simulink model "EMT"  (R2024b)
settings: Solver=ode5  StartTime=0.0  StopTime=1500  FixedStep=0.002  RelTol=1e-3
PreLoadFcn:
  | parameter;
InitFcn:
  | parameter;
StopFcn:
  | save('result.mat');
values from neighbouring files (symbols this model uses):
  A = 7.3    [parameter.m]
  a11 = (1+k1)*(1+k2)/k1/k2/iq    (= 1.54241568346)    [parameter.m]
  a11_L = a11    (= 1.54241568346)    [parameter.m]
  a12 = -(1+k1+k2)*(1+k3)/k1/k2    (= -3.86074191629)    [parameter.m]
  a12_L = a11*(1+k3+k4)/(1+k3)    (= 2.43173643789)    [parameter.m]
  a21 = -(1+k2)/k1/iq    (= -1.04963112005)    [parameter.m]
  a22 = (1+k1+k2)/k1    (= 2.46948356808)    [parameter.m]
  B = 2.71    [parameter.m]
  b11 = 0    [parameter.m]
  b12 = (1+k3)    (= 3.33)    [parameter.m]
  b21 = (1+k2)/iq    (= 2.23571428571)    [parameter.m]
  b22 = -k2    (= -2.13)    [parameter.m]
  C1_shift = 200    [parameter.m]
  Cb = 70    [parameter.m]
  Cd = 0.6    [parameter.m]
  eff_generator = eff_motor    [parameter.m]
  eff_motor = [0.80 0.80 0.84 0.84 0.83 0.85 0.83 0.83 0.83 0.80 0.80 0.80 ... (first row only)    [parameter.m]
  ele_map = [10.00,11.46,14.13,19.24,20.94,23.21,20.29,20.23,22.28,17.66,16.24,18.95,20.79,16.98,18.22,16.52,18.29,20.67,20.82,23.14,23.36,21.30,17.71,20.26,19.53,21.18,23.13,22.79,19.35,16.77,20.50,19.02,20.56,21.90,23.91,20.40,18.45,22.70,22.38,22.48,21.84,17.76,20.13,22.61,19.35,19.36,21.56,20.37,18.38,17.96,18.38,17.24,18.99,22.31,23.50,18.24,22.11,20.73,20.35,18.91,22.88,20.92,18.75,16.85,21.94,17.80,19. ...(+2007 chars)    [parameter.m]
  Fb_max = 5.5*mass    (= 247500)    [parameter.m]
  ic = 4.42    [parameter.m]
  JA = 0.4    [parameter.m]
  JB = JA    (= 0.4)    [parameter.m]
  Jc3r4 = 1e-2    (= 0.01)    [parameter.m]
  Je = 2.5    [parameter.m]
  Jh = 1e-2    (= 0.01)    [parameter.m]
  kh = 2.88    [parameter.m]
  kt = 1.83    [parameter.m]
  L = 4.472    [parameter.m]
  mass = 45000    [parameter.m]
  miu_max = 0.8    [parameter.m]
  n_generator = n_motor    [parameter.m]
  n_motor = [0 0.1 0.25 0.4 0.55 0.7 0.85 1 1.15 1.3 1.45 2.2]*3185    [parameter.m]
  nA_map = [-6000:50:-3250 -3200 0 3200 3250:50:6000]    [parameter.m]    (also in plot_result.m = [-7000:50:-3250 -3200 0 3200 3250:50:7000])
  nA_max = max(nA_map)    [parameter.m]
  nA_min = min(nA_map)    [parameter.m]
  nB_map = nA_map    [parameter.m]    (also in plot_result.m = [-7000:50:-3250 -3200 0 3200 3250:50:7000])
  nB_max = nA_max    [parameter.m]
  nB_min = nA_min    [parameter.m]
  ne_idl = 3000    [parameter.m]
  ne_map = [1600,1700,1800,1900,2000,2100,2200,2300,2400,2500,2600,2700,2800,2900,3000,3100,3200,3300,3400,3500,3600,3700,3800,3900,4000,4100,4200,4500]    [parameter.m]
  ne_max = 4200    [parameter.m]
  ne_min = 1600    [parameter.m]
  ne_start = 200    [parameter.m]
  nZ_map = [-8000:50:-4850 -4800 0 4800 4850:50:8000]    [parameter.m]
  Pb_epr = [-45 -45 -40 -30 0 30 40 45 45]    [parameter.m]
  Pb_max = [0 40 45 45 45]    [parameter.m]
  Pb_min = [-45 -45 -45 -40 0]    [parameter.m]
  Pe_ass = 210+20    (= 230)    [parameter.m]
  Pe_max = 1103    [parameter.m]
  PN0 = 0    [parameter.m]
  R_map = [0.90 0.89 0.90 0.91 0.92 0.93 0.94 0.95 0.96 0.97 0.98]/10    [parameter.m]
  rz = 0.318    [parameter.m]
  SOC0 = 60    [parameter.m]
  SOC_epr = [30 31 50 59 60 61 70 79 80]    [parameter.m]
  SOC_map = 0:10:100    [parameter.m]
  T_generator = T_motor    [parameter.m]
  T_motor = [0 0.3 0.8 1.3 1.8 2.3 2.8]/1.8*1110    [parameter.m]
  TA_max_map = [370*9549./(6000:-50:3250) 1110 1110 1110 370*9549./(3250:50:6000)]    [parameter.m]    (also in plot_result.m = [370*9549./(7000:-50:3250) 1100 1100 1100 370*9549./(3250:50)
  TA_min_map = -TA_max_map    [parameter.m]
  TAf = 0    [parameter.m]
  TB_max_map = TA_max_map    [parameter.m]    (also in plot_result.m = [370*9549./(7000:-50:3250) 1110 1110 1110 370*9549./(3250:50)
  TB_min_map = TA_min_map    [parameter.m]
  TBf = TAf    (= 0)    [parameter.m]
  Te_map = [0,599,798,998,1168,1324,1495,1660,1822,1970,2106,2235,2355,2458,2508,2543,2565,2606,2613,2649,2658,2689,2701,2707,2719,2724,2728,2740,2743,2754]    [parameter.m]
  Te_max_map = [1168,1324,1495,1660,1822,1970,2106,2235,2355,2458,2543,2606,2658,2701,2728,2743,2754,2743,2740,2724,2719,2707,2689,2649,2613,2565,2508,998]    [parameter.m]
  Te_start = 1600    [parameter.m]
  Tef = 100    [parameter.m]
  Time = 0:0.1:200    [parameter.m]
  Time_ele = 0:4:1600    [parameter.m]
  TS_A = 0.2    [parameter.m]
  TS_B = TS_A    (= 0.2)    [parameter.m]
  TS_C0 = 0.2    [parameter.m]
  TS_C1 = 0.2    [parameter.m]
  Ts_e = 0.1    [parameter.m]
  TS_Z1 = 0.2    [parameter.m]
  TS_Z2 = 0.2    [parameter.m]
  TZ_max_map = [450*9549./(8000:-50:4850) 1000 1000 1000 450*9549./(4850:50:8000)]    [parameter.m]
  TZ_min_map = -TZ_max_map    [parameter.m]
  Uoc_map = [3.258,3.668,3.733,3.783,3.833,3.877,3.912,3.941,3.973,4.013,4.200]*250    [parameter.m]
  v_cyc = 0.*(0<=Time&Time<11)+(3.75.*Time-41.25).*(11<=Time&Time<15)+15.*(15<=Time&Time<23)+(-3.*Time+84).*(23<=Time&Time<28)+0.*(28<=Time&Time<49)+(8.*Time/3-392/3).*(49<=Time&Time<61)+32.*(61<=Time&Time<85)+(-32.*Time/11+3072/11).*(85<=Time&Time<96)+0.*(96<=Time&Time<117)+(25.*Time/13-2925/13).*(117<=Time&Time<143)+50.*(143<=Time&Time<155)+(-15.*Time/8+2725/8).*(155<=Time&Time<163)+35.*(163<=Time&Time<17 ...(+70 chars)    [parameter.m]
  V_Shift12 = 32    [parameter.m]
  V_Shift21 = 25    [parameter.m]
  Voltage_epr = [750 760 900 1000 1050]    [parameter.m]
  Y_engine = 0.955    [parameter.m]
  Yc = 0.98    [parameter.m]
  Yh = 0.96    [parameter.m]
  Z1_shift = 200    [parameter.m]
  Z2_shift = 200    [parameter.m]
undefined symbols (not defined in the file or in its folder): sigbuilder_block
libraries: fl_lib x82, nesl_utility x55, simulink x49, sdl_lib x10, simulink_need_slupdate x6, powerlib_extras x1
(part 5 of 6)

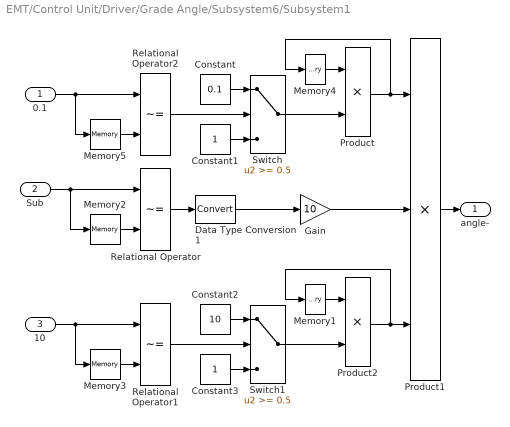
== system EMT/Control Unit/Driver/Grade Angle/Subsystem6/Subsystem1 ==
  0.1 : Inport
  Sub : Inport  Port=2
  10 : Inport  Port=3
  Constant : Constant  Value=0.1
  Constant1 : Constant
  Constant2 : Constant  Value=10
  Constant3 : Constant
  Data Type Conversion1 : DataTypeConversion  SaturateOnIntegerOverflow=off  RndMeth=Floor
  Gain : Gain  Gain=10
  Memory1 : Memory  InitialCondition=1
  Memory2 : Memory
  Memory3 : Memory
  Memory4 : Memory  InitialCondition=1
  Memory5 : Memory
  Product : Product  RndMeth=Zero
  Product1 : Product  Inputs=3  RndMeth=Zero
  Product2 : Product  RndMeth=Zero
  Relational Operator : RelationalOperator  Operator=~=  OutDataTypeStr=boolean  InputSameDT=off
  Relational Operator1 : RelationalOperator  Operator=~=  OutDataTypeStr=boolean  InputSameDT=off
  Relational Operator2 : RelationalOperator  Operator=~=  OutDataTypeStr=boolean  InputSameDT=off
  Switch : Switch  Threshold=0.5  SaturateOnIntegerOverflow=off  InputSameDT=off
  Switch1 : Switch  Threshold=0.5  SaturateOnIntegerOverflow=off  InputSameDT=off
  angle- : Outport
  wires:
  Switch1/1 -> Product2/2
  Constant3/1 -> Switch1/3
  Constant2/1 -> Switch1/1
  10/1 -> Memory3/1, Relational Operator1/1
  Relational Operator1/1 -> Switch1/2
  Memory3/1 -> Relational Operator1/2
  Memory1/1 -> Product2/1
  Product2/1 -> Product1/3, Memory1/1
  Product1/1 -> angle-/1
  Switch/1 -> Product/2
  Constant1/1 -> Switch/3
  Constant/1 -> Switch/1
  0.1/1 -> Relational Operator2/1, Memory5/1
  Relational Operator2/1 -> Switch/2
  Memory5/1 -> Relational Operator2/2
  Memory4/1 -> Product/1
  Product/1 -> Product1/1, Memory4/1
  Data Type Conversion1/1 -> Gain/1
  Relational Operator/1 -> Data Type Conversion1/1
  Sub/1 -> Memory2/1, Relational Operator/1
  Memory2/1 -> Relational Operator/2
  Gain/1 -> Product1/2

== system EMT/Control Unit/Driver/Ground Resistance Coefficient/Road/Subsystem ==
  In : Inport
  Add : Sum  Inputs=+++
  Compare To Constant1 : simulink/Logic and Bit Operations/Compare To Constant  relop=>  const=0.01  OutDataTypeStr=uint8
  Compare To Constant2 : simulink/Logic and Bit Operations/Compare To Constant  relop=>  const=0.2  OutDataTypeStr=uint8
  Compare To Constant3 : simulink/Logic and Bit Operations/Compare To Constant  relop=>  const=0.8  OutDataTypeStr=uint8
  Compare To Constant4 : simulink/Logic and Bit Operations/Compare To Constant  relop=<  const=1  OutDataTypeStr=uint8
  Data Type Conversion : DataTypeConversion  SaturateOnIntegerOverflow=off  RndMeth=Floor
  Logical Operator1 : Logic  Operator=OR  AllPortsSameDT=off  OutDataTypeStr=boolean
  Memory2 : Memory
  Judge : Outport
  wires:
  Compare To Constant2/1 -> Add/2
  Data Type Conversion/1 -> Judge/1
  Compare To Constant1/1 -> Add/1
  Add/1 -> Data Type Conversion/1
  In/1 -> Compare To Constant3/1, Compare To Constant2/1, Compare To Constant1/1
  [v_act] -> Memory2/1
  Memory2/1 -> Compare To Constant4/1
  Compare To Constant4/1 -> Logical Operator1/2
  Compare To Constant3/1 -> Logical Operator1/1
  Logical Operator1/1 -> Add/3

== system EMT/Control Unit/Driver/Ground Resistance Coefficient/Road/Subsystem1 ==
  Constant5 : Constant  Value=0.6
  Out1 : Outport
  wires:
  Constant5/1 -> Out1/1

== system EMT/Control Unit/Driver/Ground Resistance Coefficient/Road/Subsystem2 ==
  In1 : Inport
  1-D Lookup Table : Lookup_n-D  NumberOfTableDimensions=1  BreakpointsForDimension1=[-1 0 0.1 0.2 0.8 1]  Table=[0.6 0.1 0.04 0 0 0]  RndMeth=Simplest
  Saturation : Saturate  UpperLimit=1  LowerLimit=-1
  Out1 : Outport
  wires:
  Saturation/1 -> 1-D Lookup Table/1
  In1/1 -> Saturation/1
  1-D Lookup Table/1 -> Out1/1

== system EMT/Control Unit/Driver/Ground Resistance Coefficient/Road/Subsystem3 ==
  Constant1 : Constant  Value=0
  Out1 : Outport
  wires:
  Constant1/1 -> Out1/1

== system EMT/Control Unit/Driver/Ground Resistance Coefficient/Road/Subsystem4 ==
  Constant1 : Constant  Value=-0.04
  Out1 : Outport
  wires:
  Constant1/1 -> Out1/1

== system EMT/Control Unit/Driver/Ground Resistance Coefficient/Subsystem2/Subsystem4 ==
  11 : Constant
  21 : Constant  Value=2
  22 : Constant  Value=3
  31 : Constant  Value=4
  0.1 : Outport
  0.01 : Outport  Port=2
  10 : Outport  Port=3
  100 : Outport  Port=4
  wires:
  11/1 -> 0.1/1
  21/1 -> 0.01/1
  22/1 -> 10/1
  31/1 -> 100/1

== system EMT/Control Unit/Driver/Ground Resistance Coefficient/Subsystem2/Subsystem6 ==
  11 : Constant
  21 : Constant  Value=2
  22 : Constant  Value=3
  31 : Constant  Value=4
  1 : Outport
  2 : Outport  Port=2
  3 : Outport  Port=3
  4 : Outport  Port=4
  wires:
  31/1 -> 4/1
  22/1 -> 3/1
  21/1 -> 2/1
  11/1 -> 1/1

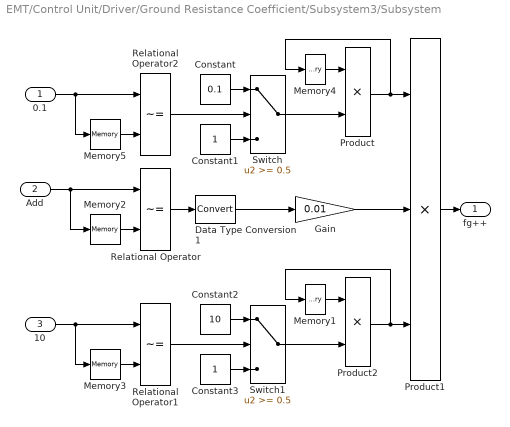
== system EMT/Control Unit/Driver/Ground Resistance Coefficient/Subsystem3/Subsystem ==
  0.1 : Inport
  Add : Inport  Port=2
  10 : Inport  Port=3
  Constant : Constant  Value=0.1
  Constant1 : Constant
  Constant2 : Constant  Value=10
  Constant3 : Constant
  Data Type Conversion1 : DataTypeConversion  SaturateOnIntegerOverflow=off  RndMeth=Floor
  Gain : Gain  Gain=0.01
  Memory1 : Memory  InitialCondition=1
  Memory2 : Memory
  Memory3 : Memory
  Memory4 : Memory  InitialCondition=1
  Memory5 : Memory
  Product : Product  RndMeth=Zero
  Product1 : Product  Inputs=3  RndMeth=Zero
  Product2 : Product  RndMeth=Zero
  Relational Operator : RelationalOperator  Operator=~=  OutDataTypeStr=boolean  InputSameDT=off
  Relational Operator1 : RelationalOperator  Operator=~=  OutDataTypeStr=boolean  InputSameDT=off
  Relational Operator2 : RelationalOperator  Operator=~=  OutDataTypeStr=boolean  InputSameDT=off
  Switch : Switch  Threshold=0.5  SaturateOnIntegerOverflow=off  InputSameDT=off
  Switch1 : Switch  Threshold=0.5  SaturateOnIntegerOverflow=off  InputSameDT=off
  fg++ : Outport
  wires:
  Gain/1 -> Product1/2
  Switch1/1 -> Product2/2
  Constant3/1 -> Switch1/3
  Constant2/1 -> Switch1/1
  10/1 -> Memory3/1, Relational Operator1/1
  Relational Operator1/1 -> Switch1/2
  Memory3/1 -> Relational Operator1/2
  Memory1/1 -> Product2/1
  Product2/1 -> Product1/3, Memory1/1
  Product1/1 -> fg++/1
  Switch/1 -> Product/2
  Constant1/1 -> Switch/3
  Constant/1 -> Switch/1
  0.1/1 -> Relational Operator2/1, Memory5/1
  Relational Operator2/1 -> Switch/2
  Memory5/1 -> Relational Operator2/2
  Memory4/1 -> Product/1
  Product/1 -> Product1/1, Memory4/1
  Data Type Conversion1/1 -> Gain/1
  Relational Operator/1 -> Data Type Conversion1/1
  Add/1 -> Memory2/1, Relational Operator/1
  Memory2/1 -> Relational Operator/2

== system EMT/Control Unit/Driver/Ground Resistance Coefficient/Subsystem3/Subsystem1 ==
  0.1 : Inport
  Sub : Inport  Port=2
  10 : Inport  Port=3
  Constant : Constant  Value=0.1
  Constant1 : Constant
  Constant2 : Constant  Value=10
  Constant3 : Constant
  Data Type Conversion1 : DataTypeConversion  SaturateOnIntegerOverflow=off  RndMeth=Floor
  Gain : Gain  Gain=0.01
  Memory1 : Memory  InitialCondition=1
  Memory2 : Memory
  Memory3 : Memory
  Memory4 : Memory  InitialCondition=1
  Memory5 : Memory
  Product : Product  RndMeth=Zero
  Product1 : Product  Inputs=3  RndMeth=Zero
  Product2 : Product  RndMeth=Zero
  Relational Operator : RelationalOperator  Operator=~=  OutDataTypeStr=boolean  InputSameDT=off
  Relational Operator1 : RelationalOperator  Operator=~=  OutDataTypeStr=boolean  InputSameDT=off
  Relational Operator2 : RelationalOperator  Operator=~=  OutDataTypeStr=boolean  InputSameDT=off
  Switch : Switch  Threshold=0.5  SaturateOnIntegerOverflow=off  InputSameDT=off
  Switch1 : Switch  Threshold=0.5  SaturateOnIntegerOverflow=off  InputSameDT=off
  fg-- : Outport
  wires:
  Gain/1 -> Product1/2
  Memory2/1 -> Relational Operator/2
  Sub/1 -> Relational Operator/1, Memory2/1
  Relational Operator/1 -> Data Type Conversion1/1
  Data Type Conversion1/1 -> Gain/1
  Product/1 -> Memory4/1, Product1/1
  Memory4/1 -> Product/1
  Memory5/1 -> Relational Operator2/2
  Relational Operator2/1 -> Switch/2
  0.1/1 -> Memory5/1, Relational Operator2/1
  Constant/1 -> Switch/1
  Constant1/1 -> Switch/3
  Switch/1 -> Product/2
  Product1/1 -> fg--/1
  Product2/1 -> Memory1/1, Product1/3
  Memory1/1 -> Product2/1
  Memory3/1 -> Relational Operator1/2
  Relational Operator1/1 -> Switch1/2
  10/1 -> Relational Operator1/1, Memory3/1
  Constant2/1 -> Switch1/1
  Constant3/1 -> Switch1/3
  Switch1/1 -> Product2/2

== system EMT/Control Unit/Driver/Pedal /Subsystem13/Subsystem4 ==
  11 : Constant
  21 : Constant  Value=2
  22 : Constant  Value=3
  31 : Constant  Value=4
  0.1 : Outport
  0.01 : Outport  Port=2
  10 : Outport  Port=3
  100 : Outport  Port=4
  wires:
  31/1 -> 100/1
  22/1 -> 10/1
  21/1 -> 0.01/1
  11/1 -> 0.1/1

== system EMT/Control Unit/Driver/Pedal /Subsystem13/Subsystem6 ==
  11 : Constant
  21 : Constant  Value=2
  22 : Constant  Value=3
  31 : Constant  Value=4
  1 : Outport
  2 : Outport  Port=2
  3 : Outport  Port=3
  4 : Outport  Port=4
  wires:
  11/1 -> 1/1
  21/1 -> 2/1
  22/1 -> 3/1
  31/1 -> 4/1

== system EMT/Control Unit/Driver/Pedal /Subsystem5/Subsystem ==
  0.1 : Inport
  Add : Inport  Port=2
  10 : Inport  Port=3
  Constant : Constant  Value=0.1
  Constant1 : Constant
  Constant2 : Constant  Value=10
  Constant3 : Constant
  Data Type Conversion1 : DataTypeConversion  SaturateOnIntegerOverflow=off  RndMeth=Floor
  Gain : Gain  Gain=0.1
  Memory1 : Memory  InitialCondition=1
  Memory2 : Memory
  Memory3 : Memory
  Memory4 : Memory  InitialCondition=1
  Memory5 : Memory
  Product : Product  RndMeth=Zero
  Product1 : Product  Inputs=3  RndMeth=Zero
  Product2 : Product  RndMeth=Zero
  Relational Operator : RelationalOperator  Operator=~=  OutDataTypeStr=boolean  InputSameDT=off
  Relational Operator1 : RelationalOperator  Operator=~=  OutDataTypeStr=boolean  InputSameDT=off
  Relational Operator2 : RelationalOperator  Operator=~=  OutDataTypeStr=boolean  InputSameDT=off
  Switch : Switch  Threshold=0.5  SaturateOnIntegerOverflow=off  InputSameDT=off
  Switch1 : Switch  Threshold=0.5  SaturateOnIntegerOverflow=off  InputSameDT=off
  pedal++ : Outport
  wires:
  Memory2/1 -> Relational Operator/2
  Add/1 -> Relational Operator/1, Memory2/1
  Relational Operator/1 -> Data Type Conversion1/1
  Data Type Conversion1/1 -> Gain/1
  Product/1 -> Memory4/1, Product1/1
  Memory4/1 -> Product/1
  Memory5/1 -> Relational Operator2/2
  Relational Operator2/1 -> Switch/2
  0.1/1 -> Memory5/1, Relational Operator2/1
  Constant/1 -> Switch/1
  Constant1/1 -> Switch/3
  Switch/1 -> Product/2
  Product1/1 -> pedal++/1
  Product2/1 -> Memory1/1, Product1/3
  Memory1/1 -> Product2/1
  Memory3/1 -> Relational Operator1/2
  Relational Operator1/1 -> Switch1/2
  10/1 -> Relational Operator1/1, Memory3/1
  Constant2/1 -> Switch1/1
  Constant3/1 -> Switch1/3
  Switch1/1 -> Product2/2
  Gain/1 -> Product1/2

== system EMT/Control Unit/Driver/Pedal /Subsystem5/Subsystem1 ==
  0.1 : Inport
  Sub : Inport  Port=2
  10 : Inport  Port=3
  Constant : Constant  Value=0.1
  Constant1 : Constant
  Constant2 : Constant  Value=10
  Constant3 : Constant
  Data Type Conversion1 : DataTypeConversion  SaturateOnIntegerOverflow=off  RndMeth=Floor
  Gain : Gain  Gain=0.1
  Memory1 : Memory  InitialCondition=1
  Memory2 : Memory
  Memory3 : Memory
  Memory4 : Memory  InitialCondition=1
  Memory5 : Memory
  Product : Product  RndMeth=Zero
  Product1 : Product  Inputs=3  RndMeth=Zero
  Product2 : Product  RndMeth=Zero
  Relational Operator : RelationalOperator  Operator=~=  OutDataTypeStr=boolean  InputSameDT=off
  Relational Operator1 : RelationalOperator  Operator=~=  OutDataTypeStr=boolean  InputSameDT=off
  Relational Operator2 : RelationalOperator  Operator=~=  OutDataTypeStr=boolean  InputSameDT=off
  Switch : Switch  Threshold=0.5  SaturateOnIntegerOverflow=off  InputSameDT=off
  Switch1 : Switch  Threshold=0.5  SaturateOnIntegerOverflow=off  InputSameDT=off
  pedal-- : Outport
  wires:
  Switch1/1 -> Product2/2
  Constant3/1 -> Switch1/3
  Constant2/1 -> Switch1/1
  10/1 -> Memory3/1, Relational Operator1/1
  Relational Operator1/1 -> Switch1/2
  Memory3/1 -> Relational Operator1/2
  Memory1/1 -> Product2/1
  Product2/1 -> Product1/3, Memory1/1
  Product1/1 -> pedal--/1
  Switch/1 -> Product/2
  Constant1/1 -> Switch/3
  Constant/1 -> Switch/1
  0.1/1 -> Relational Operator2/1, Memory5/1
  Relational Operator2/1 -> Switch/2
  Memory5/1 -> Relational Operator2/2
  Memory4/1 -> Product/1
  Product/1 -> Product1/1, Memory4/1
  Data Type Conversion1/1 -> Gain/1
  Relational Operator/1 -> Data Type Conversion1/1
  Sub/1 -> Memory2/1, Relational Operator/1
  Memory2/1 -> Relational Operator/2
  Gain/1 -> Product1/2

== system EMT/Control Unit/Driver/Wheel Angle/Subsystem1/Subsystem4 ==
  11 : Constant
  21 : Constant  Value=2
  22 : Constant  Value=3
  31 : Constant  Value=4
  0.1 : Outport
  0.01 : Outport  Port=2
  10 : Outport  Port=3
  100 : Outport  Port=4
  wires:
  31/1 -> 100/1
  22/1 -> 10/1
  21/1 -> 0.01/1
  11/1 -> 0.1/1

== system EMT/Control Unit/Driver/Wheel Angle/Subsystem1/Subsystem6 ==
  11 : Constant
  21 : Constant  Value=2
  22 : Constant  Value=3
  31 : Constant  Value=4
  1 : Outport
  2 : Outport  Port=2
  3 : Outport  Port=3
  4 : Outport  Port=4
  wires:
  11/1 -> 1/1
  21/1 -> 2/1
  22/1 -> 3/1
  31/1 -> 4/1

== system EMT/Control Unit/Driver/Wheel Angle/Subsystem2/Subsystem ==
  0.1 : Inport
  Add : Inport  Port=2
  10 : Inport  Port=3
  Constant : Constant  Value=0.1
  Constant1 : Constant
  Constant2 : Constant  Value=10
  Constant3 : Constant
  Data Type Conversion1 : DataTypeConversion  SaturateOnIntegerOverflow=off  RndMeth=Floor
  Gain : Gain
  Memory1 : Memory  InitialCondition=1
  Memory2 : Memory
  Memory3 : Memory
  Memory4 : Memory  InitialCondition=1
  Memory5 : Memory
  Product : Product  RndMeth=Zero
  Product1 : Product  Inputs=3  RndMeth=Zero
  Product2 : Product  RndMeth=Zero
  Relational Operator : RelationalOperator  Operator=~=  OutDataTypeStr=boolean  InputSameDT=off
  Relational Operator1 : RelationalOperator  Operator=~=  OutDataTypeStr=boolean  InputSameDT=off
  Relational Operator2 : RelationalOperator  Operator=~=  OutDataTypeStr=boolean  InputSameDT=off
  Switch : Switch  Threshold=0.5  SaturateOnIntegerOverflow=off  InputSameDT=off
  Switch1 : Switch  Threshold=0.5  SaturateOnIntegerOverflow=off  InputSameDT=off
  wheel++ : Outport
  wires:
  Memory2/1 -> Relational Operator/2
  Add/1 -> Relational Operator/1, Memory2/1
  Relational Operator/1 -> Data Type Conversion1/1
  Data Type Conversion1/1 -> Gain/1
  Product/1 -> Memory4/1, Product1/1
  Memory4/1 -> Product/1
  Memory5/1 -> Relational Operator2/2
  Relational Operator2/1 -> Switch/2
  0.1/1 -> Memory5/1, Relational Operator2/1
  Constant/1 -> Switch/1
  Constant1/1 -> Switch/3
  Switch/1 -> Product/2
  Product1/1 -> wheel++/1
  Product2/1 -> Memory1/1, Product1/3
  Memory1/1 -> Product2/1
  Memory3/1 -> Relational Operator1/2
  Relational Operator1/1 -> Switch1/2
  10/1 -> Relational Operator1/1, Memory3/1
  Constant2/1 -> Switch1/1
  Constant3/1 -> Switch1/3
  Switch1/1 -> Product2/2
  Gain/1 -> Product1/2

== system EMT/Control Unit/Driver/Wheel Angle/Subsystem2/Subsystem1 ==
  0.1 : Inport
  Sub : Inport  Port=2
  10 : Inport  Port=3
  Constant : Constant  Value=0.1
  Constant1 : Constant
  Constant2 : Constant  Value=10
  Constant3 : Constant
  Data Type Conversion1 : DataTypeConversion  SaturateOnIntegerOverflow=off  RndMeth=Floor
  Gain : Gain
  Memory1 : Memory  InitialCondition=1
  Memory2 : Memory
  Memory3 : Memory
  Memory4 : Memory  InitialCondition=1
  Memory5 : Memory
  Product : Product  RndMeth=Zero
  Product1 : Product  Inputs=3  RndMeth=Zero
  Product2 : Product  RndMeth=Zero
  Relational Operator : RelationalOperator  Operator=~=  OutDataTypeStr=boolean  InputSameDT=off
  Relational Operator1 : RelationalOperator  Operator=~=  OutDataTypeStr=boolean  InputSameDT=off
  Relational Operator2 : RelationalOperator  Operator=~=  OutDataTypeStr=boolean  InputSameDT=off
  Switch : Switch  Threshold=0.5  SaturateOnIntegerOverflow=off  InputSameDT=off
  Switch1 : Switch  Threshold=0.5  SaturateOnIntegerOverflow=off  InputSameDT=off
  wheel-- : Outport
  wires:
  Switch1/1 -> Product2/2
  Constant3/1 -> Switch1/3
  Constant2/1 -> Switch1/1
  10/1 -> Memory3/1, Relational Operator1/1
  Relational Operator1/1 -> Switch1/2
  Memory3/1 -> Relational Operator1/2
  Memory1/1 -> Product2/1
  Product2/1 -> Product1/3, Memory1/1
  Product1/1 -> wheel--/1
  Switch/1 -> Product/2
  Constant1/1 -> Switch/3
  Constant/1 -> Switch/1
  0.1/1 -> Relational Operator2/1, Memory5/1
  Relational Operator2/1 -> Switch/2
  Memory5/1 -> Relational Operator2/2
  Memory4/1 -> Product/1
  Product/1 -> Product1/1, Memory4/1
  Data Type Conversion1/1 -> Gain/1
  Relational Operator/1 -> Data Type Conversion1/1
  Sub/1 -> Memory2/1, Relational Operator/1
  Memory2/1 -> Relational Operator/2
  Gain/1 -> Product1/2

== system EMT/Power Coupler /Z1/Z/Power/Speed Sensor ==
  Ideal Rotational Motion Sensor : fl_lib/Mechanical/Mechanical Sensors/Ideal Rotational Motion Sensor  reference=foundation.enum.MeasurementReference.difference  acceleration_port=false  velocity_port=true  position_port=true  wrap_angle=false  offset=0 rad
  PS-Simulink Converter : nesl_utility/PS-Simulink Converter  PhysicalDomain=network_engine_domain  SubClassName=ps_output  LeftPortType=input  RightPortType=output  PseudoPeriodic=off  Frequencies=[]  VectorFormat=1-D array  Unit=rad/s  AffineConversion=off
  Reference : fl_lib/Mechanical/Rotational Elements/Mechanical Rotational Reference
  Tire Radius2 : Gain  Gain=30/pi
  shaft : PMIOPort  Side=Left
  r/min : Outport
  wires:
  Tire Radius2/1 -> r/min/1
  PS-Simulink Converter/1 -> Tire Radius2/1
  connections:
  shaft/RConn1 -- Ideal Rotational Motion Sensor/LConn1
  Reference/LConn1 -- Ideal Rotational Motion Sensor/RConn1
  PS-Simulink Converter/LConn1 -- Ideal Rotational Motion Sensor/RConn2

== system EMT/Power Coupler /Z1/Z/Power/Torque Sensor ==
  Ideal Torque Sensor : fl_lib/Mechanical/Mechanical Sensors/Ideal Torque Sensor
  PS-Simulink Converter : nesl_utility/PS-Simulink Converter  PhysicalDomain=network_engine_domain  SubClassName=ps_output  LeftPortType=input  RightPortType=output  PseudoPeriodic=off  Frequencies=[]  VectorFormat=1-D array  Unit=1  AffineConversion=off
  In : PMIOPort  Side=Left
  Out : PMIOPort  Port=2  Side=Right
  Nm : Outport
  wires:
  PS-Simulink Converter/1 -> Nm/1
  connections:
  PS-Simulink Converter/LConn1 -- Ideal Torque Sensor/RConn2
  In/RConn1 -- Ideal Torque Sensor/LConn1
  Ideal Torque Sensor/RConn1 -- Out/RConn1

== system EMT/Power Coupler /Z1/Z/Power1/Speed Sensor ==
  Ideal Rotational Motion Sensor : fl_lib/Mechanical/Mechanical Sensors/Ideal Rotational Motion Sensor  reference=foundation.enum.MeasurementReference.difference  acceleration_port=false  velocity_port=true  position_port=true  wrap_angle=false  offset=0 rad
  PS-Simulink Converter : nesl_utility/PS-Simulink Converter  PhysicalDomain=network_engine_domain  SubClassName=ps_output  LeftPortType=input  RightPortType=output  PseudoPeriodic=off  Frequencies=[]  VectorFormat=1-D array  Unit=rad/s  AffineConversion=off
  Reference : fl_lib/Mechanical/Rotational Elements/Mechanical Rotational Reference
  Tire Radius2 : Gain  Gain=30/pi
  shaft : PMIOPort  Side=Left
  r/min : Outport
  wires:
  PS-Simulink Converter/1 -> Tire Radius2/1
  Tire Radius2/1 -> r/min/1
  connections:
  PS-Simulink Converter/LConn1 -- Ideal Rotational Motion Sensor/RConn2
  Reference/LConn1 -- Ideal Rotational Motion Sensor/RConn1
  shaft/RConn1 -- Ideal Rotational Motion Sensor/LConn1

== system EMT/Power Coupler /Z1/Z/Power1/Torque Sensor ==
  Ideal Torque Sensor : fl_lib/Mechanical/Mechanical Sensors/Ideal Torque Sensor
  PS-Simulink Converter : nesl_utility/PS-Simulink Converter  PhysicalDomain=network_engine_domain  SubClassName=ps_output  LeftPortType=input  RightPortType=output  PseudoPeriodic=off  Frequencies=[]  VectorFormat=1-D array  Unit=1  AffineConversion=off
  In : PMIOPort  Side=Left
  Out : PMIOPort  Port=2  Side=Right
  Nm : Outport
  wires:
  PS-Simulink Converter/1 -> Nm/1
  connections:
  Ideal Torque Sensor/RConn1 -- Out/RConn1
  In/RConn1 -- Ideal Torque Sensor/LConn1
  PS-Simulink Converter/LConn1 -- Ideal Torque Sensor/RConn2

== system EMT/Power Coupler /Z1/Z/Z1/Slip Sensor ==
  Abs : Abs  SaturateOnIntegerOverflow=off
  Ideal Rotational Motion Sensor : fl_lib/Mechanical/Mechanical Sensors/Ideal Rotational Motion Sensor  reference=foundation.enum.MeasurementReference.difference  acceleration_port=false  velocity_port=true  position_port=true  wrap_angle=false  offset=0 rad
  PS-Simulink Converter : nesl_utility/PS-Simulink Converter  PhysicalDomain=network_engine_domain  SubClassName=ps_output  LeftPortType=input  RightPortType=output  PseudoPeriodic=off  Frequencies=[]  VectorFormat=1-D array  Unit=1  AffineConversion=off
  Tire Radius2 : Gain  Gain=30/pi
  In : PMIOPort  Side=Left
  Out : PMIOPort  Port=2  Side=Right
  r/min : Outport
  wires:
  PS-Simulink Converter/1 -> Tire Radius2/1
  Tire Radius2/1 -> Abs/1
  Abs/1 -> r/min/1
  connections:
  PS-Simulink Converter/LConn1 -- Ideal Rotational Motion Sensor/RConn2
  Out/RConn1 -- Ideal Rotational Motion Sensor/RConn1
  In/RConn1 -- Ideal Rotational Motion Sensor/LConn1

== system EMT/Power Coupler /Z2/Z/Power/Speed Sensor ==
  Ideal Rotational Motion Sensor : fl_lib/Mechanical/Mechanical Sensors/Ideal Rotational Motion Sensor  reference=foundation.enum.MeasurementReference.difference  acceleration_port=false  velocity_port=true  position_port=true  wrap_angle=false  offset=0 rad
  PS-Simulink Converter : nesl_utility/PS-Simulink Converter  PhysicalDomain=network_engine_domain  SubClassName=ps_output  LeftPortType=input  RightPortType=output  PseudoPeriodic=off  Frequencies=[]  VectorFormat=1-D array  Unit=rad/s  AffineConversion=off
  Reference : fl_lib/Mechanical/Rotational Elements/Mechanical Rotational Reference
  Tire Radius2 : Gain  Gain=30/pi
  shaft : PMIOPort  Side=Left
  r/min : Outport
  wires:
  Tire Radius2/1 -> r/min/1
  PS-Simulink Converter/1 -> Tire Radius2/1
  connections:
  shaft/RConn1 -- Ideal Rotational Motion Sensor/LConn1
  Reference/LConn1 -- Ideal Rotational Motion Sensor/RConn1
  PS-Simulink Converter/LConn1 -- Ideal Rotational Motion Sensor/RConn2

== system EMT/Power Coupler /Z2/Z/Power/Torque Sensor ==
  Ideal Torque Sensor : fl_lib/Mechanical/Mechanical Sensors/Ideal Torque Sensor
  PS-Simulink Converter : nesl_utility/PS-Simulink Converter  PhysicalDomain=network_engine_domain  SubClassName=ps_output  LeftPortType=input  RightPortType=output  PseudoPeriodic=off  Frequencies=[]  VectorFormat=1-D array  Unit=1  AffineConversion=off
  In : PMIOPort  Side=Left
  Out : PMIOPort  Port=2  Side=Right
  Nm : Outport
  wires:
  PS-Simulink Converter/1 -> Nm/1
  connections:
  PS-Simulink Converter/LConn1 -- Ideal Torque Sensor/RConn2
  In/RConn1 -- Ideal Torque Sensor/LConn1
  Ideal Torque Sensor/RConn1 -- Out/RConn1

== system EMT/Power Coupler /Z2/Z/Power1/Speed Sensor ==
  Ideal Rotational Motion Sensor : fl_lib/Mechanical/Mechanical Sensors/Ideal Rotational Motion Sensor  reference=foundation.enum.MeasurementReference.difference  acceleration_port=false  velocity_port=true  position_port=true  wrap_angle=false  offset=0 rad
  PS-Simulink Converter : nesl_utility/PS-Simulink Converter  PhysicalDomain=network_engine_domain  SubClassName=ps_output  LeftPortType=input  RightPortType=output  PseudoPeriodic=off  Frequencies=[]  VectorFormat=1-D array  Unit=rad/s  AffineConversion=off
  Reference : fl_lib/Mechanical/Rotational Elements/Mechanical Rotational Reference
  Tire Radius2 : Gain  Gain=30/pi
  shaft : PMIOPort  Side=Left
  r/min : Outport
  wires:
  PS-Simulink Converter/1 -> Tire Radius2/1
  Tire Radius2/1 -> r/min/1
  connections:
  PS-Simulink Converter/LConn1 -- Ideal Rotational Motion Sensor/RConn2
  Reference/LConn1 -- Ideal Rotational Motion Sensor/RConn1
  shaft/RConn1 -- Ideal Rotational Motion Sensor/LConn1

== system EMT/Power Coupler /Z2/Z/Power1/Torque Sensor ==
  Ideal Torque Sensor : fl_lib/Mechanical/Mechanical Sensors/Ideal Torque Sensor
  PS-Simulink Converter : nesl_utility/PS-Simulink Converter  PhysicalDomain=network_engine_domain  SubClassName=ps_output  LeftPortType=input  RightPortType=output  PseudoPeriodic=off  Frequencies=[]  VectorFormat=1-D array  Unit=1  AffineConversion=off
  In : PMIOPort  Side=Left
  Out : PMIOPort  Port=2  Side=Right
  Nm : Outport
  wires:
  PS-Simulink Converter/1 -> Nm/1
  connections:
  Ideal Torque Sensor/RConn1 -- Out/RConn1
  In/RConn1 -- Ideal Torque Sensor/LConn1
  PS-Simulink Converter/LConn1 -- Ideal Torque Sensor/RConn2

== system EMT/Power Coupler /Z2/Z/Z2/Slip Sensor ==
  Abs : Abs  SaturateOnIntegerOverflow=off
  Ideal Rotational Motion Sensor : fl_lib/Mechanical/Mechanical Sensors/Ideal Rotational Motion Sensor  reference=foundation.enum.MeasurementReference.difference  acceleration_port=false  velocity_port=true  position_port=true  wrap_angle=false  offset=0 rad
  PS-Simulink Converter : nesl_utility/PS-Simulink Converter  PhysicalDomain=network_engine_domain  SubClassName=ps_output  LeftPortType=input  RightPortType=output  PseudoPeriodic=off  Frequencies=[]  VectorFormat=1-D array  Unit=1  AffineConversion=off
  Tire Radius2 : Gain  Gain=30/pi
  In : PMIOPort  Side=Left
  Out : PMIOPort  Port=2  Side=Right
  r/min : Outport
  wires:
  PS-Simulink Converter/1 -> Tire Radius2/1
  Tire Radius2/1 -> Abs/1
  Abs/1 -> r/min/1
  connections:
  PS-Simulink Converter/LConn1 -- Ideal Rotational Motion Sensor/RConn2
  Out/RConn1 -- Ideal Rotational Motion Sensor/RConn1
  In/RConn1 -- Ideal Rotational Motion Sensor/LConn1

== system EMT/motorA/Motor/Mechanical Body/Resistance/Torque Actuator ==
  torque : Inport
  Ideal Torque Source : fl_lib/Mechanical/Mechanical Sources/Ideal Torque Source
  Mechanical Rotational Reference : fl_lib/Mechanical/Rotational Elements/Mechanical Rotational Reference
  Simulink-PS Converter : nesl_utility/Simulink-PS Converter  PhysicalDomain=network_engine_domain  SubClassName=ps_input  LeftPortType=input  RightPortType=output  PseudoPeriodic=off  Frequencies=[]  NoiseDistribution=none  NoiseParameters=[]  Unit=N*m  AffineConversion=off  FilteringAndDerivatives=zero  SimscapeFilterOrder=1  InputFilterTimeConstant=.001  UdotUserProvided=0
  shaft : PMIOPort  Side=Right
  wires:
  torque/1 -> Simulink-PS Converter/1
  connections:
  shaft/RConn1 -- Ideal Torque Source/LConn1
  Mechanical Rotational Reference/LConn1 -- Ideal Torque Source/RConn2
  Simulink-PS Converter/RConn1 -- Ideal Torque Source/RConn1

== system EMT/motorB/Motor/Mechanical Body/Resistance/Torque Actuator ==
  torque : Inport
  Ideal Torque Source : fl_lib/Mechanical/Mechanical Sources/Ideal Torque Source
  Mechanical Rotational Reference : fl_lib/Mechanical/Rotational Elements/Mechanical Rotational Reference
  Simulink-PS Converter : nesl_utility/Simulink-PS Converter  PhysicalDomain=network_engine_domain  SubClassName=ps_input  LeftPortType=input  RightPortType=output  PseudoPeriodic=off  Frequencies=[]  NoiseDistribution=none  NoiseParameters=[]  Unit=N*m  AffineConversion=off  FilteringAndDerivatives=filter  SimscapeFilterOrder=1  InputFilterTimeConstant=.001  UdotUserProvided=1
  shaft : PMIOPort  Side=Right
  wires:
  torque/1 -> Simulink-PS Converter/1
  connections:
  shaft/RConn1 -- Ideal Torque Source/LConn1
  Mechanical Rotational Reference/LConn1 -- Ideal Torque Source/RConn2
  Simulink-PS Converter/RConn1 -- Ideal Torque Source/RConn1

== system EMT/Control Unit/Control/Power Distribution/Feasible Control Range/State Calculation/Speed ==
  stage : Inport
  ne : Inport  Port=2
  no : Inport  Port=3
  Demux1 : Demux  Outputs=2
  Z : Subsystem
  nA : Outport
  nB : Outport  Port=2
  wires:
  Demux1/2 -> nB/1
  Demux1/1 -> nA/1
  stage/1 -> Z/1(s)
  ne/1 -> Z/2(ne)
  no/1 -> Z/3(no)
  Z/1(nAnB) -> Demux1/1

== system EMT/Control Unit/Control/Power Distribution/Feasible Control Range/State Calculation/Subsystem3 ==
  0 : Inport
  Constant : Constant
  Constant1 : Constant  Value=4
  MinMax : MinMax  Function=max  Inputs=2
  MinMax1 : MinMax  Inputs=2
  1 : Outport
  wires:
  0/1 -> MinMax/1
  Constant/1 -> MinMax/2
  MinMax/1 -> MinMax1/1
  Constant1/1 -> MinMax1/2
  MinMax1/1 -> 1/1

== system EMT/Control Unit/Control/Power Distribution/Feasible Control Range/State Predition/TA Range ==
  nA : Inport
  Lookup Table : Lookup  InputValues=nA_map  Table=TA_max_map  SaturateOnIntegerOverflow=off
  Lookup Table1 : Lookup  InputValues=nA_map  Table=TA_min_map  SaturateOnIntegerOverflow=off
  Mux1 : Mux  Inputs=2
  Saturation1 : Saturate  UpperLimit=max(nA_map)  LowerLimit=min(nA_map)
  Saturation2 : Saturate  UpperLimit=max(nA_map)  LowerLimit=min(nA_map)
  TA_R : Outport
  wires:
  Mux1/1 -> TA_R/1
  Saturation2/1 -> Lookup Table1/1
  Saturation1/1 -> Lookup Table/1
  Lookup Table1/1 -> Mux1/2  "TA_min"
  Lookup Table/1 -> Mux1/1  "TA_max"
  nA/1 -> Saturation1/1, Saturation2/1

== system EMT/Control Unit/Control/Power Distribution/Feasible Control Range/State Predition/TB Range ==
  nB : Inport
  Lookup Table : Lookup  InputValues=nB_map  Table=TB_max_map  SaturateOnIntegerOverflow=off
  Lookup Table1 : Lookup  InputValues=nB_map  Table=TB_min_map  SaturateOnIntegerOverflow=off
  Mux1 : Mux  Inputs=2
  Saturation1 : Saturate  UpperLimit=max(nB_map)  LowerLimit=min(nB_map)
  Saturation2 : Saturate  UpperLimit=max(nB_map)  LowerLimit=min(nB_map)
  TB_R : Outport
  wires:
  Mux1/1 -> TB_R/1
  Lookup Table1/1 -> Mux1/2  "TB_min"
  Lookup Table/1 -> Mux1/1  "TB_max"
  nB/1 -> Saturation2/1, Saturation1/1
  Saturation1/1 -> Lookup Table/1
  Saturation2/1 -> Lookup Table1/1

== system EMT/Control Unit/Control/Power Distribution/Feasible Control Range/State Predition/Te Range ==
  ne_act : Inport
  Constant : Constant  Value=0
  Lookup Table : Lookup  InputValues=ne_map  Table=Te_max_map  SaturateOnIntegerOverflow=off
  Mux1 : Mux  Inputs=2
  Saturation1 : Saturate  UpperLimit=max(ne_map)  LowerLimit=min(ne_map)
  Te_k : Outport
  wires:
  Mux1/1 -> Te_k/1
  ne_act/1 -> Saturation1/1
  Saturation1/1 -> Lookup Table/1
  Constant/1 -> Mux1/2  "Te_min"
  Lookup Table/1 -> Mux1/1  "Te_max"

== system EMT/Control Unit/Control/Power Distribution/Feasible Control Range/State Predition/Z ==
  stage : Inport
  ne_act : Inport  Port=2
  no_act : Inport  Port=3
  Mux2 : Mux  Inputs=3
  Saturation1 : Saturate  UpperLimit=ne_max  LowerLimit=ne_min
  Saturation2 : Saturate  UpperLimit=ne_max  LowerLimit=ne_min
  ne Range : Subsystem
  ne_k : Outport
  wires:
  Saturation2/1 -> Mux2/3
  Saturation1/1 -> Mux2/2
  ne_act/1 -> Mux2/1
  ne Range/1(ne_max) -> Saturation1/1
  ne Range/2(ne_min) -> Saturation2/1
  Mux2/1 -> ne_k/1
  stage/1 -> ne Range/1(stage)
  no_act/1 -> ne Range/2(no)

== system EMT/Control Unit/Control/Prepare Stage/motorA torque/TA_com1/Subsystem1 ==
  nA_act : Inport
  Constant : Constant  Value=a11*(ne_idl+100)
  Memory5 : Memory
  Subsystem : Subsystem
  Sum1 : Sum  Inputs=+-
  TA_com : Outport
  wires:
  Constant/1 -> Sum1/1
  Memory5/1 -> Sum1/2
  nA_act/1 -> Memory5/1
  Sum1/1 -> Subsystem/1(dnA)
  Subsystem/1(TA) -> TA_com/1

== system EMT/Control Unit/Control/Prepare Stage/motorA torque/TA_com1/Subsystem2 ==
  PN : Inport
  nA : Inport  Port=2
  Fcn : Fcn  Expr=abs(9549*u(1)/u(2))/2
  Memory5 : Memory
  Mux : Mux  Inputs=2
  Subsystem : Subsystem
  TA_com : Outport
  wires:
  Memory5/1 -> Subsystem/1(0)
  Subsystem/1(1) -> Mux/2
  Mux/1 -> Fcn/1
  nA/1 -> Memory5/1
  PN/1 -> Mux/1
  Fcn/1 -> TA_com/1

== system EMT/Control Unit/Control/Shift Stage/EVT2->EVT1/motorZ torque/Subsystem1 ==
  nZ_act : Inport
  Constant3 : Constant  Value=0
  Memory5 : Memory
  PID Controller2 : simulink_need_slupdate/PID Controller  P=2  I=0.01  D=0.1
  Sum1 : Sum  Inputs=+-
  TZ_com : Outport
  wires:
  Memory5/1 -> Sum1/2
  Constant3/1 -> Sum1/1
  nZ_act/1 -> Memory5/1
  Sum1/1 -> PID Controller2/1
  PID Controller2/1 -> TZ_com/1

== system EMT/Control Unit/Control/Power Distribution/Feasible Control Range/State Calculation/Speed/Z ==
  s : Inport
  ne : Inport  Port=2
  no : Inport  Port=3
  Multiport Switch1 : MultiPortSwitch  Inputs=4  SaturateOnIntegerOverflow=off  InputSameDT=off
  Mux2 : Mux  Inputs=2
  Subsystem2 : Subsystem
  Subsystem3 : Subsystem
  Subsystem4 : Subsystem
  Subsystem5 : Subsystem
  nAnB : Outport
  wires:
  no/1 -> Mux2/2
  ne/1 -> Mux2/1
  s/1 -> Multiport Switch1/1
  Multiport Switch1/1 -> nAnB/1
  Mux2/1 -> Subsystem3/1(neno), Subsystem4/1(neno), Subsystem5/1(neno), Subsystem2/1(neno)
  Subsystem5/1(nAnB) -> Multiport Switch1/4
  Subsystem4/1(nAnB) -> Multiport Switch1/3
  Subsystem3/1(nAnB) -> Multiport Switch1/2
  Subsystem2/1(nAnB) -> Multiport Switch1/5

== system EMT/Control Unit/Control/Power Distribution/Feasible Control Range/State Predition/Z/ne Range ==
  stage : Inport
  no : Inport  Port=2
  Demux : Demux  Outputs=2
  Multiport Switch : MultiPortSwitch  Inputs=4  SaturateOnIntegerOverflow=off  InputSameDT=off
  Subsystem : Subsystem
  Subsystem1 : Subsystem
  Subsystem2 : Subsystem
  Subsystem3 : Subsystem
  Subsystem4 : Subsystem
  ne_max : Outport
  ne_min : Outport  Port=2
  wires:
  Subsystem4/1(ne) -> Multiport Switch/5
  Subsystem3/1(1) -> Multiport Switch/1
  Subsystem/1(ne) -> Multiport Switch/2
  Subsystem1/1(ne) -> Multiport Switch/3
  Subsystem2/1(ne) -> Multiport Switch/4
  Multiport Switch/1 -> Demux/1
  Demux/1 -> ne_max/1
  Demux/2 -> ne_min/1
  stage/1 -> Subsystem3/1(0)
  no/1 -> Subsystem/1(no), Subsystem4/1(no), Subsystem2/1(no), Subsystem1/1(no)

== system EMT/Control Unit/Control/Prepare Stage/motorA torque/TA_com1/Subsystem1/Subsystem ==
  dnA : Inport
  Abs : Abs  SaturateOnIntegerOverflow=off
  Constant1 : Constant  Value=min(TA_min_map)
  Constant2 : Constant  Value=max(TA_max_map)
  PID Controller2 : simulink_need_slupdate/PID Controller  P=10  I=0.1  D=1
  Switch1 : Switch  Criteria=u2 > Threshold  Threshold=1000  SaturateOnIntegerOverflow=off  InputSameDT=off
  Switch2 : Switch  Criteria=u2 > Threshold  SaturateOnIntegerOverflow=off  InputSameDT=off
  TA : Outport
  wires:
  dnA/1 -> PID Controller2/1, Switch2/2, Abs/1
  PID Controller2/1 -> Switch1/3
  Switch1/1 -> TA/1
  Abs/1 -> Switch1/2
  Switch2/1 -> Switch1/1
  Constant1/1 -> Switch2/3
  Constant2/1 -> Switch2/1

== system EMT/Control Unit/Control/Prepare Stage/motorA torque/TA_com1/Subsystem2/Subsystem ==
  0 : Inport
  Constant : Constant
  Switch : Switch  Criteria=u2 ~= 0  SaturateOnIntegerOverflow=off  InputSameDT=off
  1 : Outport
  wires:
  Constant/1 -> Switch/3
  0/1 -> Switch/2, Switch/1
  Switch/1 -> 1/1

== system EMT/Control Unit/Control/Power Distribution/Feasible Control Range/State Calculation/Speed/Z/Subsystem2 ==
  neno : Inport
  Mux2 : Mux  Inputs=2
  ne_max1 : Fcn  Expr=b11/kt*u(1)+b12*u(2)
  ne_max3 : Fcn  Expr=a11_L*u(1)+a12*u(2)
  nAnB : Outport
  wires:
  ne_max3/1 -> Mux2/1
  ne_max1/1 -> Mux2/2
  neno/1 -> ne_max1/1, ne_max3/1
  Mux2/1 -> nAnB/1

== system EMT/Control Unit/Control/Power Distribution/Feasible Control Range/State Calculation/Speed/Z/Subsystem3 ==
  neno : Inport
  Mux2 : Mux  Inputs=2
  ne_max1 : Fcn  Expr=b11*u(1)+b12*u(2)
  ne_max3 : Fcn  Expr=a11*u(1)+a12*u(2)
  nAnB : Outport
  wires:
  ne_max3/1 -> Mux2/1
  ne_max1/1 -> Mux2/2
  neno/1 -> ne_max1/1, ne_max3/1
  Mux2/1 -> nAnB/1

== system EMT/Control Unit/Control/Power Distribution/Feasible Control Range/State Calculation/Speed/Z/Subsystem4 ==
  neno : Inport
  Mux2 : Mux  Inputs=2
  ne_max1 : Fcn  Expr=b11*u(1)+b12*u(2)
  ne_max3 : Fcn  Expr=a11*u(1)+a12*u(2)
  nAnB : Outport
  wires:
  Mux2/1 -> nAnB/1
  neno/1 -> ne_max3/1, ne_max1/1
  ne_max1/1 -> Mux2/2
  ne_max3/1 -> Mux2/1

== system EMT/Control Unit/Control/Power Distribution/Feasible Control Range/State Calculation/Speed/Z/Subsystem5 ==
  neno : Inport
  Mux2 : Mux  Inputs=2
  ne_max1 : Fcn  Expr=b21*u(1)+b22*u(2)
  ne_max3 : Fcn  Expr=a21*u(1)+a22*u(2)
  nAnB : Outport
  wires:
  ne_max3/1 -> Mux2/1
  ne_max1/1 -> Mux2/2
  neno/1 -> ne_max1/1, ne_max3/1
  Mux2/1 -> nAnB/1

== system EMT/Control Unit/Control/Power Distribution/Feasible Control Range/State Predition/Z/ne Range/Subsystem ==
  no : Inport
  Mux2 : Mux  Inputs=2
  ne_max : Fcn  Expr=(nA_max-a12*u)/a11
  ne_min : Fcn  Expr=(nA_min-a12*u)/a11
  ne : Outport
  wires:
  no/1 -> ne_min/1, ne_max/1
  ne_max/1 -> Mux2/1
  Mux2/1 -> ne/1
  ne_min/1 -> Mux2/2

== system EMT/Control Unit/Control/Power Distribution/Feasible Control Range/State Predition/Z/ne Range/Subsystem1 ==
  no : Inport
  Mux2 : Mux  Inputs=2
  ne_max : Fcn  Expr=(nB_max-b22*u)/b21
  ne_min : Fcn  Expr=(nA_min-a12*u)/a11
  ne : Outport
  wires:
  ne_min/1 -> Mux2/2
  Mux2/1 -> ne/1
  ne_max/1 -> Mux2/1
  no/1 -> ne_max/1, ne_min/1

== system EMT/Control Unit/Control/Power Distribution/Feasible Control Range/State Predition/Z/ne Range/Subsystem2 ==
  no : Inport
  MinMax1 : MinMax  Inputs=2
  MinMax2 : MinMax  Function=max  Inputs=2
  Mux2 : Mux  Inputs=2
  ne_max1 : Fcn  Expr=(nA_min-a22*u)/a21
  ne_max2 : Fcn  Expr=(nB_max-b22*u)/b21
  ne_min1 : Fcn  Expr=(nA_max-a22*u)/a21
  ne_min2 : Fcn  Expr=(nB_min-b22*u)/b21
  ne : Outport
  wires:
  MinMax2/1 -> Mux2/2
  MinMax1/1 -> Mux2/1
  no/1 -> ne_max1/1, ne_min1/1, ne_min2/1, ne_max2/1
  Mux2/1 -> ne/1
  ne_max1/1 -> MinMax1/1
  ne_max2/1 -> MinMax1/2
  ne_min1/1 -> MinMax2/1
  ne_min2/1 -> MinMax2/2

== system EMT/Control Unit/Control/Power Distribution/Feasible Control Range/State Predition/Z/ne Range/Subsystem3 ==
  0 : Inport
  Constant : Constant
  Constant1 : Constant  Value=4
  MinMax : MinMax  Function=max  Inputs=2
  MinMax1 : MinMax  Inputs=2
  1 : Outport
  wires:
  0/1 -> MinMax/1
  Constant/1 -> MinMax/2
  MinMax/1 -> MinMax1/1
  Constant1/1 -> MinMax1/2
  MinMax1/1 -> 1/1

== system EMT/Control Unit/Control/Power Distribution/Feasible Control Range/State Predition/Z/ne Range/Subsystem4 ==
  no : Inport
  Mux2 : Mux  Inputs=2
  ne_max : Fcn  Expr=(nA_max-a12_L*u)/a11_L
  ne_min : Fcn  Expr=(nA_min-a12_L*u)/a11_L
  ne : Outport
  wires:
  ne_min/1 -> Mux2/2
  Mux2/1 -> ne/1
  ne_max/1 -> Mux2/1
  no/1 -> ne_max/1, ne_min/1
